simulink model "G474_Mode2_Direct_Start_Repair"  (R2024b)
settings: Solver=FixedStepDiscrete  StartTime=0.0  StopTime=q.stop_time  FixedStep=p.Ts  RelTol=1e-3
InitFcn:
  | m2_project_root=fileparts(fileparts(get_param(bdroot,'FileName')));Simulink.fileGenControl('set','CacheFolder',fullfile(m2_project_root,'work'),'CodeGenFolder',fullfile(m2_project_root,'work'),'createDir',true);m2_ws=get_param(bdroot,'ModelWorkspace');m2_q=getVariable(m2_ws,'q');if isfield(m2_q,'random_initial_angle') && m2_q.random_initial_angle,m2_q.initial_theta_e=2*pi*rand();end;m2_q.initial_state=[0;0;m2_q.initial_rpm*2*pi/60;m2_q.initial_theta_e];assignin(m2_ws,'q',m2_q);fprintf('MODE2 physical initial electrical angle: %.9f deg (random=%d)\n',m2_q.initial_theta_e*180/pi,m2_q.random_initial_angle);
model workspace (MAT data in the model file):
  fSin = [0 0.00153398001567 0.00306795700453 0.00460192607716 0.00613588513806 0.00766982883215 0.00920375529677 0.0107376594096 0.0122715383768 0.0138053894043 0.0153392059729 0.0168729871511 ... (1025 elements, 1025x1)]
  p : object (value not decoded)
  q : object (value not decoded)
  s0 : object (value not decoded)
symbols that are objects in the model workspace (value not decoded): p, q, s0
(part 2 of 2)

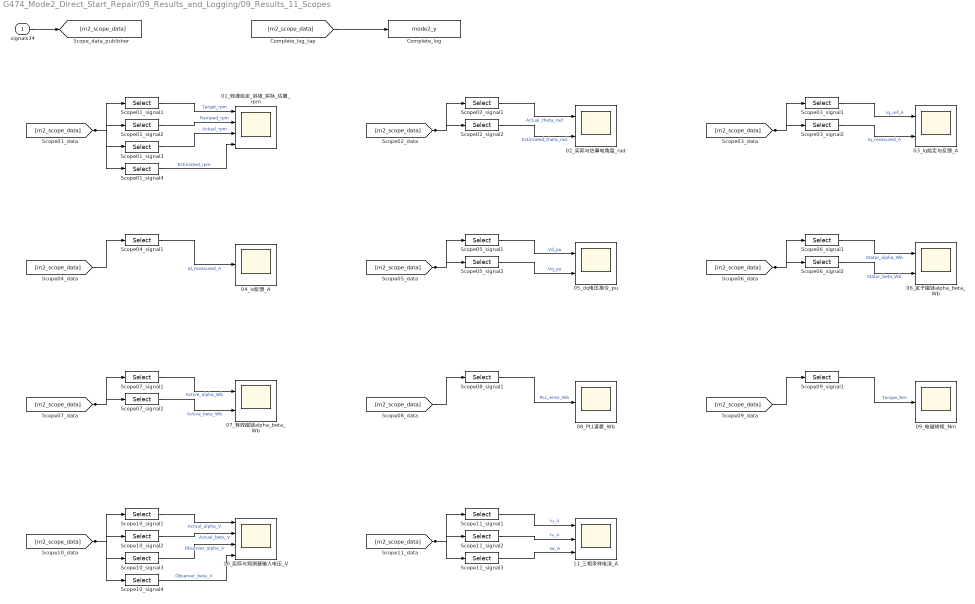
== system G474_Mode2_Direct_Start_Repair/09_Results_and_Logging/09_Results_11_Scopes ==
  signals34 : Inport
  01_转速给定_斜坡_实际_估算_rpm : Scope  NumInputPorts=4
  02_实际与估算电角度_rad : Scope  NumInputPorts=2
  03_Iq给定与反馈_A : Scope  NumInputPorts=2
  04_Id反馈_A : Scope
  05_dq电压指令_pu : Scope  NumInputPorts=2
  06_定子磁链alpha_beta_Wb : Scope  NumInputPorts=2
  07_有效磁链alpha_beta_Wb : Scope  NumInputPorts=2
  08_PLL误差_Wb : Scope
  09_电磁转矩_Nm : Scope
  10_实际与观测器输入电压_V : Scope  NumInputPorts=4
  11_三相采样电流_A : Scope  NumInputPorts=3
  Complete_log : ToWorkspace  VariableName=mode2_y  SaveFormat=Timeseries  SampleTime=-1
  Scope01_signal1 : Selector  InputPortWidth=34  IndexOptions=Index vector (dialog)  Indices=31  OutputSizes=1
  Scope01_signal2 : Selector  InputPortWidth=34  IndexOptions=Index vector (dialog)  Indices=23  OutputSizes=1
  Scope01_signal3 : Selector  InputPortWidth=34  IndexOptions=Index vector (dialog)  Indices=12  OutputSizes=1
  Scope01_signal4 : Selector  InputPortWidth=34  IndexOptions=Index vector (dialog)  Indices=3  OutputSizes=1
  Scope02_signal1 : Selector  InputPortWidth=34  IndexOptions=Index vector (dialog)  Indices=13  OutputSizes=1
  Scope02_signal2 : Selector  InputPortWidth=34  IndexOptions=Index vector (dialog)  Indices=1  OutputSizes=1
  Scope03_signal1 : Selector  InputPortWidth=34  IndexOptions=Index vector (dialog)  Indices=22  OutputSizes=1
  Scope03_signal2 : Selector  InputPortWidth=34  IndexOptions=Index vector (dialog)  Indices=19  OutputSizes=1
  Scope04_signal1 : Selector  InputPortWidth=34  IndexOptions=Index vector (dialog)  Indices=18  OutputSizes=1
  Scope05_signal1 : Selector  InputPortWidth=34  IndexOptions=Index vector (dialog)  Indices=20  OutputSizes=1
  Scope05_signal2 : Selector  InputPortWidth=34  IndexOptions=Index vector (dialog)  Indices=21  OutputSizes=1
  Scope06_signal1 : Selector  InputPortWidth=34  IndexOptions=Index vector (dialog)  Indices=6  OutputSizes=1
  Scope06_signal2 : Selector  InputPortWidth=34  IndexOptions=Index vector (dialog)  Indices=7  OutputSizes=1
  Scope07_signal1 : Selector  InputPortWidth=34  IndexOptions=Index vector (dialog)  Indices=4  OutputSizes=1
  Scope07_signal2 : Selector  InputPortWidth=34  IndexOptions=Index vector (dialog)  Indices=5  OutputSizes=1
  Scope08_signal1 : Selector  InputPortWidth=34  IndexOptions=Index vector (dialog)  Indices=8  OutputSizes=1
  Scope09_signal1 : Selector  InputPortWidth=34  IndexOptions=Index vector (dialog)  Indices=14  OutputSizes=1
  Scope10_signal1 : Selector  InputPortWidth=34  IndexOptions=Index vector (dialog)  Indices=26  OutputSizes=1
  Scope10_signal2 : Selector  InputPortWidth=34  IndexOptions=Index vector (dialog)  Indices=27  OutputSizes=1
  Scope10_signal3 : Selector  InputPortWidth=34  IndexOptions=Index vector (dialog)  Indices=10  OutputSizes=1
  Scope10_signal4 : Selector  InputPortWidth=34  IndexOptions=Index vector (dialog)  Indices=11  OutputSizes=1
  Scope11_signal1 : Selector  InputPortWidth=34  IndexOptions=Index vector (dialog)  Indices=15  OutputSizes=1
  Scope11_signal2 : Selector  InputPortWidth=34  IndexOptions=Index vector (dialog)  Indices=16  OutputSizes=1
  Scope11_signal3 : Selector  InputPortWidth=34  IndexOptions=Index vector (dialog)  Indices=17  OutputSizes=1
  wires:
  signals34/1 -> [m2_scope_data]
  [m2_scope_data] -> Complete_log/1
  [m2_scope_data] -> Scope01_signal1/1, Scope01_signal2/1, Scope01_signal3/1, Scope01_signal4/1
  Scope01_signal1/1 -> 01_转速给定_斜坡_实际_估算_rpm/1  "Target_rpm"
  Scope01_signal2/1 -> 01_转速给定_斜坡_实际_估算_rpm/2  "Ramped_rpm"
  Scope01_signal3/1 -> 01_转速给定_斜坡_实际_估算_rpm/3  "Actual_rpm"
  Scope01_signal4/1 -> 01_转速给定_斜坡_实际_估算_rpm/4  "Estimated_rpm"
  [m2_scope_data] -> Scope02_signal1/1, Scope02_signal2/1
  Scope02_signal1/1 -> 02_实际与估算电角度_rad/1  "Actual_theta_rad"
  Scope02_signal2/1 -> 02_实际与估算电角度_rad/2  "Estimated_theta_rad"
  [m2_scope_data] -> Scope03_signal1/1, Scope03_signal2/1
  Scope03_signal1/1 -> 03_Iq给定与反馈_A/1  "Iq_ref_A"
  Scope03_signal2/1 -> 03_Iq给定与反馈_A/2  "Iq_measured_A"
  [m2_scope_data] -> Scope04_signal1/1
  Scope04_signal1/1 -> 04_Id反馈_A/1  "Id_measured_A"
  [m2_scope_data] -> Scope05_signal1/1, Scope05_signal2/1
  Scope05_signal1/1 -> 05_dq电压指令_pu/1  "Vd_pu"
  Scope05_signal2/1 -> 05_dq电压指令_pu/2  "Vq_pu"
  [m2_scope_data] -> Scope06_signal1/1, Scope06_signal2/1
  Scope06_signal1/1 -> 06_定子磁链alpha_beta_Wb/1  "Stator_alpha_Wb"
  Scope06_signal2/1 -> 06_定子磁链alpha_beta_Wb/2  "Stator_beta_Wb"
  [m2_scope_data] -> Scope07_signal1/1, Scope07_signal2/1
  Scope07_signal1/1 -> 07_有效磁链alpha_beta_Wb/1  "Active_alpha_Wb"
  Scope07_signal2/1 -> 07_有效磁链alpha_beta_Wb/2  "Active_beta_Wb"
  [m2_scope_data] -> Scope08_signal1/1
  Scope08_signal1/1 -> 08_PLL误差_Wb/1  "PLL_error_Wb"
  [m2_scope_data] -> Scope09_signal1/1
  Scope09_signal1/1 -> 09_电磁转矩_Nm/1  "Torque_Nm"
  [m2_scope_data] -> Scope10_signal1/1, Scope10_signal2/1, Scope10_signal3/1, Scope10_signal4/1
  Scope10_signal1/1 -> 10_实际与观测器输入电压_V/1  "Actual_alpha_V"
  Scope10_signal2/1 -> 10_实际与观测器输入电压_V/2  "Actual_beta_V"
  Scope10_signal3/1 -> 10_实际与观测器输入电压_V/3  "Observer_alpha_V"
  Scope10_signal4/1 -> 10_实际与观测器输入电压_V/4  "Observer_beta_V"
  [m2_scope_data] -> Scope11_signal1/1, Scope11_signal2/1, Scope11_signal3/1
  Scope11_signal1/1 -> 11_三相采样电流_A/1  "Iu_A"
  Scope11_signal2/1 -> 11_三相采样电流_A/2  "Iv_A"
  Scope11_signal3/1 -> 11_三相采样电流_A/3  "Iw_A"

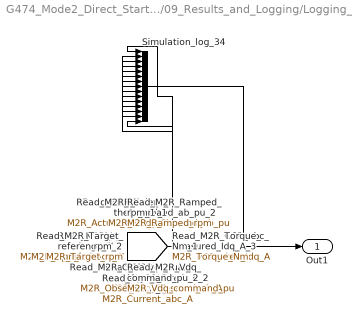
== system G474_Mode2_Direct_Start_Repair/09_Results_and_Logging/Logging_taps ==
  Simulation_log_34 : Mux  Inputs=15
  Out1 : Outport
  wires:
  [M2R_Actual_theta_rad] -> Simulation_log_34/3
  [M2R_Actual_rpm] -> Simulation_log_34/2
  [M2R_Torque_Nm] -> Simulation_log_34/4
  [M2R_CCR_abc] -> Simulation_log_34/12
  [M2R_Command_ab_pu] -> Simulation_log_34/10
  [M2R_Current_abc_A] -> Simulation_log_34/5
  [M2R_Observer_y11] -> Simulation_log_34/1
  [M2R_Iq_reference_A] -> Simulation_log_34/8
  Simulation_log_34/1 -> Out1/1
  [M2R_Vdq_command_pu] -> Simulation_log_34/7
  [M2R_Measured_Idq_A] -> Simulation_log_34/6
  [M2R_Measured_ab_A] -> Simulation_log_34/15
  [M2R_Bridge_voltage_V] -> Simulation_log_34/11
  [M2R_Target_rpm] -> Simulation_log_34/13
  [M2R_Mode_2] -> Simulation_log_34/14
  [M2R_Ramped_rpm] -> Simulation_log_34/9

== system G474_Mode2_Direct_Start_Repair/03_Hybrid_Flux_Observer/02_Active_Flux_Models/Current model ==
  theta_previous : Inport
  Id : Inport  Port=2
  Active scalar : Sum
  Cos : Trigonometry  Operator=cos
  Direction : Mux  Inputs=2
  PM flux : Constant  Value=p.Flux
  Projection : Product  Inputs=**
  Saliency : Gain  Gain=p.Ld-p.Lq
  Sin : Trigonometry
  psi_I : Outport
  wires:
  Projection/1 -> psi_I/1
  Sin/1 -> Direction/2
  Active scalar/1 -> Projection/1
  Cos/1 -> Direction/1
  Saliency/1 -> Active scalar/2
  PM flux/1 -> Active scalar/1
  theta_previous/1 -> Cos/1, Sin/1
  Direction/1 -> Projection/2
  Id/1 -> Saliency/1

== system G474_Mode2_Direct_Start_Repair/03_Hybrid_Flux_Observer/02_Active_Flux_Models/Voltage model extraction ==
  psi_s_previous : Inport
  current_ab : Inport  Port=2
  Active flux : Sum  Inputs=+-
  Inductive flux : Gain  Gain=p.Lq
  psi_V : Outport
  wires:
  Active flux/1 -> psi_V/1
  Inductive flux/1 -> Active flux/2
  psi_s_previous/1 -> Active flux/1
  current_ab/1 -> Inductive flux/1

== system G474_Mode2_Direct_Start_Repair/03_Hybrid_Flux_Observer/03_Flux_Feedback/Alpha_PI ==
  note: flux.c: Comp_Interg += error*Comp_Ki; Ucomp = error*Comp_Kp + Comp_Interg.
      | No integral/output saturation in this firmware branch. SMO selection freezes PI memory.
  error : Inport
  integral_enable : Inport  Port=2
  Enable_integral : Switch  Criteria=u2 ~= 0  SaturateOnIntegerOverflow=off  InputSameDT=off
  Integral_candidate : Sum
  Integral_increment : Gain  Gain=Ki
  Pre_output : Sum
  Previous_integral : UnitDelay  SampleTime=Ts  HasFrameUpgradeWarning=on
  Proportional : Gain  Gain=Kp
  Ucomp : Outport
  integral : Outport  Port=2
  wires:
  Pre_output/1 -> Ucomp/1
  Proportional/1 -> Pre_output/1
  integral_enable/1 -> Enable_integral/2
  Integral_candidate/1 -> Enable_integral/1
  Previous_integral/1 -> Integral_candidate/1, Enable_integral/3
  Integral_increment/1 -> Integral_candidate/2
  Enable_integral/1 -> Previous_integral/1, integral/1, Pre_output/2
  error/1 -> Integral_increment/1, Proportional/1

== system G474_Mode2_Direct_Start_Repair/03_Hybrid_Flux_Observer/03_Flux_Feedback/Beta_PI ==
  note: flux.c: Comp_Interg += error*Comp_Ki; Ucomp = error*Comp_Kp + Comp_Interg.
      | No integral/output saturation in this firmware branch. SMO selection freezes PI memory.
  error : Inport
  integral_enable : Inport  Port=2
  Enable_integral : Switch  Criteria=u2 ~= 0  SaturateOnIntegerOverflow=off  InputSameDT=off
  Integral_candidate : Sum
  Integral_increment : Gain  Gain=Ki
  Pre_output : Sum
  Previous_integral : UnitDelay  SampleTime=Ts  HasFrameUpgradeWarning=on
  Proportional : Gain  Gain=Kp
  Ucomp : Outport
  integral : Outport  Port=2
  wires:
  Pre_output/1 -> Ucomp/1
  Proportional/1 -> Pre_output/1
  integral_enable/1 -> Enable_integral/2
  Integral_candidate/1 -> Enable_integral/1
  Previous_integral/1 -> Integral_candidate/1, Enable_integral/3
  Integral_increment/1 -> Integral_candidate/2
  Enable_integral/1 -> Previous_integral/1, integral/1, Pre_output/2
  error/1 -> Integral_increment/1, Proportional/1

== system G474_Mode2_Direct_Start_Repair/03_Hybrid_Flux_Observer/03_Flux_Feedback/SMO_feedback ==
  In1 : Inport
  Boundary normalization : Gain  Gain=1/p.SMO_Boundary
  Boundary saturation : Saturate  UpperLimit=1  LowerLimit=-1
  Sliding gain : Gain  Gain=p.SMO_Kslide
  Out1 : Outport
  wires:
  Sliding gain/1 -> Out1/1
  Boundary saturation/1 -> Sliding gain/1
  In1/1 -> Boundary normalization/1
  Boundary normalization/1 -> Boundary saturation/1

== system G474_Mode2_Direct_Start_Repair/03_Hybrid_Flux_Observer/05_PLL_and_Angle/PLL ==
  psi_V : Inport
  theta_previous : Inport  Port=2
  Angle_update : Subsystem
      settings: OpenFcn=open_system(gcb,'force')
      mask Display: port_label('input',1,'In1');port_label('input',2,'In2');port_label('output',1,'Out1');
  PLL_PI : Subsystem  mask{Kp=p.PLL_kp, Ki=p.PLL_ki, Ts=p.Ts}
      mask prompts: Kp "Kp (source coefficient)"; Ki "Ki (per call, already discrete)"; Ts "Execution period (s)"
      settings: OpenFcn=open_system(gcb,'force')
      mask Display: port_label('input',1,'PLL_Err');port_label('input',2,'step_limit');port_label('output',1,'PLL_Ui');port_label('output',2,'PLL_Interg');
  Phase_detector : Subsystem
      settings: OpenFcn=open_system(gcb,'force')
      mask Display: port_label('input',1,'In1');port_label('input',2,'In2');port_label('output',1,'Out1');
  Step limit value : Constant  Value=p.pll_step_limit
  theta_new : Outport
  step_rad : Outport  Port=2
  PLL_error : Outport  Port=3
  wires:
  Angle_update/1(Out1) -> theta_new/1
  Step limit value/1 -> PLL_PI/2(step_limit)
  Phase_detector/1(Out1) -> PLL_error/1, PLL_PI/1(PLL_Err)
  PLL_PI/1(PLL_Ui) -> Angle_update/2(In2), step_rad/1
  theta_previous/1 -> Angle_update/1(In1), Phase_detector/2(In2)
  psi_V/1 -> Phase_detector/1(In1)

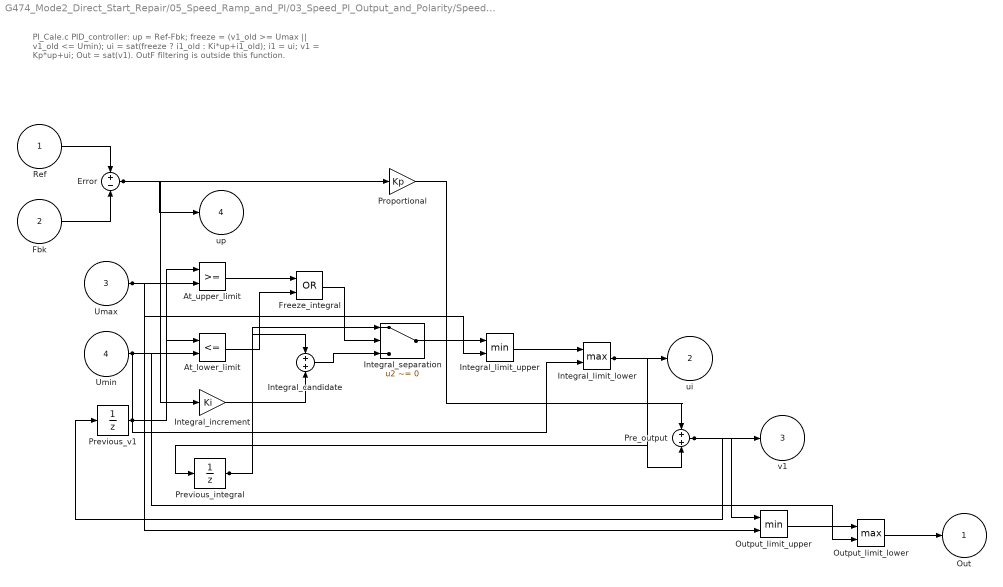
== system G474_Mode2_Direct_Start_Repair/05_Speed_Ramp_and_PI/03_Speed_PI_Output_and_Polarity/Speed_PI ==
  note: PI_Cale.c PID_controller:
      | up = Ref-Fbk; freeze = (v1_old >= Umax || v1_old <= Umin);
      | ui = sat(freeze ? i1_old : Ki*up+i1_old); i1 = ui;
      | v1 = Kp*up+ui; Out = sat(v1). OutF filtering is outside this function.
  Ref : Inport
  Fbk : Inport  Port=2
  Umax : Inport  Port=3
  Umin : Inport  Port=4
  At_lower_limit : RelationalOperator  Operator=<=  OutDataTypeStr=boolean  RndMeth=Simplest  InputSameDT=off
  At_upper_limit : RelationalOperator  OutDataTypeStr=boolean  RndMeth=Simplest  InputSameDT=off
  Error : Sum  Inputs=+-
  Freeze_integral : Logic  Operator=OR  AllPortsSameDT=off  OutDataTypeStr=boolean
  Integral_candidate : Sum
  Integral_increment : Gain  Gain=Ki
  Integral_limit_lower : MinMax  Function=max  Inputs=2
  Integral_limit_upper : MinMax  Inputs=2
  Integral_separation : Switch  Criteria=u2 ~= 0  SaturateOnIntegerOverflow=off  InputSameDT=off
  Output_limit_lower : MinMax  Function=max  Inputs=2
  Output_limit_upper : MinMax  Inputs=2
  Pre_output : Sum
  Previous_integral : UnitDelay  SampleTime=Ts  HasFrameUpgradeWarning=on
  Previous_v1 : UnitDelay  SampleTime=Ts  HasFrameUpgradeWarning=on
  Proportional : Gain  Gain=Kp
  Out : Outport
  ui : Outport  Port=2
  v1 : Outport  Port=3
  up : Outport  Port=4
  wires:
  Umax/1 -> Output_limit_upper/2, Integral_limit_upper/2, At_upper_limit/2
  Ref/1 -> Error/1
  At_lower_limit/1 -> Freeze_integral/2
  Error/1 -> Proportional/1, Integral_increment/1, up/1
  Fbk/1 -> Error/2
  At_upper_limit/1 -> Freeze_integral/1
  Umin/1 -> Integral_limit_lower/2, Output_limit_lower/2, At_lower_limit/2
  Previous_v1/1 -> At_upper_limit/1, At_lower_limit/1
  Integral_increment/1 -> Integral_candidate/2
  Previous_integral/1 -> Integral_candidate/1, Integral_separation/1
  Freeze_integral/1 -> Integral_separation/2
  Integral_candidate/1 -> Integral_separation/3
  Proportional/1 -> Pre_output/1
  Integral_separation/1 -> Integral_limit_upper/1
  Integral_limit_upper/1 -> Integral_limit_lower/1
  Integral_limit_lower/1 -> Pre_output/2, ui/1, Previous_integral/1
  Pre_output/1 -> Previous_v1/1, Output_limit_upper/1, v1/1
  Output_limit_upper/1 -> Output_limit_lower/1
  Output_limit_lower/1 -> Out/1

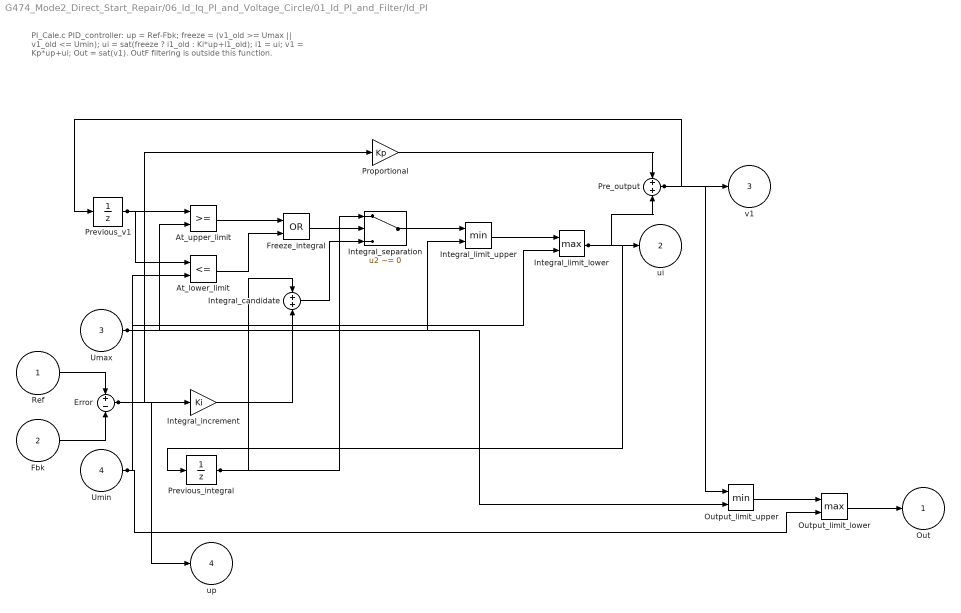
== system G474_Mode2_Direct_Start_Repair/06_Id_Iq_PI_and_Voltage_Circle/01_Id_PI_and_Filter/Id_PI ==
  note: PI_Cale.c PID_controller:
      | up = Ref-Fbk; freeze = (v1_old >= Umax || v1_old <= Umin);
      | ui = sat(freeze ? i1_old : Ki*up+i1_old); i1 = ui;
      | v1 = Kp*up+ui; Out = sat(v1). OutF filtering is outside this function.
  Ref : Inport
  Fbk : Inport  Port=2
  Umax : Inport  Port=3
  Umin : Inport  Port=4
  At_lower_limit : RelationalOperator  Operator=<=  OutDataTypeStr=boolean  RndMeth=Simplest  InputSameDT=off
  At_upper_limit : RelationalOperator  OutDataTypeStr=boolean  RndMeth=Simplest  InputSameDT=off
  Error : Sum  Inputs=+-
  Freeze_integral : Logic  Operator=OR  AllPortsSameDT=off  OutDataTypeStr=boolean
  Integral_candidate : Sum
  Integral_increment : Gain  Gain=Ki
  Integral_limit_lower : MinMax  Function=max  Inputs=2
  Integral_limit_upper : MinMax  Inputs=2
  Integral_separation : Switch  Criteria=u2 ~= 0  SaturateOnIntegerOverflow=off  InputSameDT=off
  Output_limit_lower : MinMax  Function=max  Inputs=2
  Output_limit_upper : MinMax  Inputs=2
  Pre_output : Sum
  Previous_integral : UnitDelay  SampleTime=Ts  HasFrameUpgradeWarning=on
  Previous_v1 : UnitDelay  SampleTime=Ts  HasFrameUpgradeWarning=on
  Proportional : Gain  Gain=Kp
  Out : Outport
  ui : Outport  Port=2
  v1 : Outport  Port=3
  up : Outport  Port=4
  wires:
  Umax/1 -> Output_limit_upper/2, Integral_limit_upper/2, At_upper_limit/2
  Previous_v1/1 -> At_lower_limit/1, At_upper_limit/1
  Ref/1 -> Error/1
  At_lower_limit/1 -> Freeze_integral/2
  Error/1 -> Proportional/1, Integral_increment/1, up/1
  Fbk/1 -> Error/2
  At_upper_limit/1 -> Freeze_integral/1
  Umin/1 -> Integral_limit_lower/2, Output_limit_lower/2, At_lower_limit/2
  Integral_increment/1 -> Integral_candidate/2
  Previous_integral/1 -> Integral_candidate/1, Integral_separation/1
  Freeze_integral/1 -> Integral_separation/2
  Integral_candidate/1 -> Integral_separation/3
  Proportional/1 -> Pre_output/1
  Integral_separation/1 -> Integral_limit_upper/1
  Integral_limit_upper/1 -> Integral_limit_lower/1
  Integral_limit_lower/1 -> Previous_integral/1, Pre_output/2, ui/1
  Pre_output/1 -> Previous_v1/1, Output_limit_upper/1, v1/1
  Output_limit_upper/1 -> Output_limit_lower/1
  Output_limit_lower/1 -> Out/1

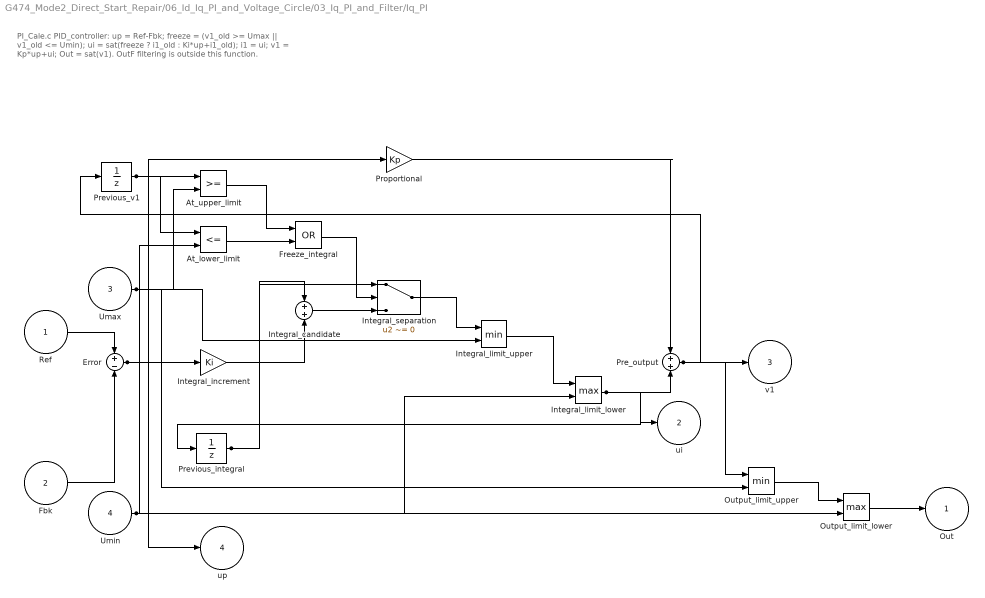
== system G474_Mode2_Direct_Start_Repair/06_Id_Iq_PI_and_Voltage_Circle/03_Iq_PI_and_Filter/Iq_PI ==
  note: PI_Cale.c PID_controller:
      | up = Ref-Fbk; freeze = (v1_old >= Umax || v1_old <= Umin);
      | ui = sat(freeze ? i1_old : Ki*up+i1_old); i1 = ui;
      | v1 = Kp*up+ui; Out = sat(v1). OutF filtering is outside this function.
  Ref : Inport
  Fbk : Inport  Port=2
  Umax : Inport  Port=3
  Umin : Inport  Port=4
  At_lower_limit : RelationalOperator  Operator=<=  OutDataTypeStr=boolean  RndMeth=Simplest  InputSameDT=off
  At_upper_limit : RelationalOperator  OutDataTypeStr=boolean  RndMeth=Simplest  InputSameDT=off
  Error : Sum  Inputs=+-
  Freeze_integral : Logic  Operator=OR  AllPortsSameDT=off  OutDataTypeStr=boolean
  Integral_candidate : Sum
  Integral_increment : Gain  Gain=Ki
  Integral_limit_lower : MinMax  Function=max  Inputs=2
  Integral_limit_upper : MinMax  Inputs=2
  Integral_separation : Switch  Criteria=u2 ~= 0  SaturateOnIntegerOverflow=off  InputSameDT=off
  Output_limit_lower : MinMax  Function=max  Inputs=2
  Output_limit_upper : MinMax  Inputs=2
  Pre_output : Sum
  Previous_integral : UnitDelay  SampleTime=Ts  HasFrameUpgradeWarning=on
  Previous_v1 : UnitDelay  SampleTime=Ts  HasFrameUpgradeWarning=on
  Proportional : Gain  Gain=Kp
  Out : Outport
  ui : Outport  Port=2
  v1 : Outport  Port=3
  up : Outport  Port=4
  wires:
  Output_limit_upper/1 -> Output_limit_lower/1
  Pre_output/1 -> Output_limit_upper/1, Previous_v1/1, v1/1
  Integral_limit_lower/1 -> ui/1, Pre_output/2, Previous_integral/1
  Integral_limit_upper/1 -> Integral_limit_lower/1
  Integral_separation/1 -> Integral_limit_upper/1
  Proportional/1 -> Pre_output/1
  Integral_candidate/1 -> Integral_separation/3
  Freeze_integral/1 -> Integral_separation/2
  Output_limit_lower/1 -> Out/1
  Previous_integral/1 -> Integral_separation/1, Integral_candidate/1
  Integral_increment/1 -> Integral_candidate/2
  Error/1 -> Integral_increment/1, up/1, Proportional/1
  At_upper_limit/1 -> Freeze_integral/1
  Previous_v1/1 -> At_lower_limit/1, At_upper_limit/1
  Umax/1 -> At_upper_limit/2, Output_limit_upper/2, Integral_limit_upper/2
  Fbk/1 -> Error/2
  Umin/1 -> Output_limit_lower/2, At_lower_limit/2, Integral_limit_lower/2
  Ref/1 -> Error/1
  At_lower_limit/1 -> Freeze_integral/2

== system G474_Mode2_Direct_Start_Repair/03_Hybrid_Flux_Observer/05_PLL_and_Angle/PLL/Angle_update ==
  In1 : Inport
  In2 : Inport  Port=2
  Angle update : Sum
  Two pi : Constant  Value=2*pi
  Wrap 2pi : Math  Operator=mod
  Out1 : Outport
  wires:
  In1/1 -> Angle update/1
  Wrap 2pi/1 -> Out1/1
  Angle update/1 -> Wrap 2pi/1
  In2/1 -> Angle update/2
  Two pi/1 -> Wrap 2pi/2

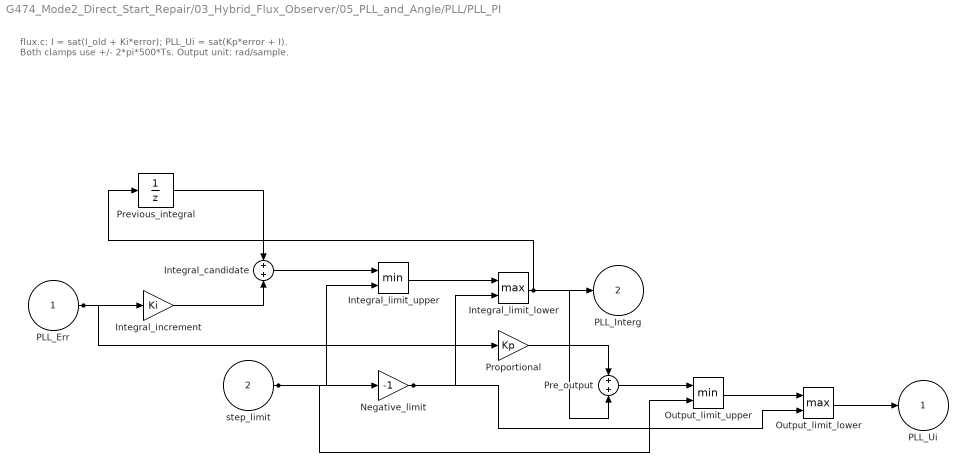
== system G474_Mode2_Direct_Start_Repair/03_Hybrid_Flux_Observer/05_PLL_and_Angle/PLL/PLL_PI ==
  note: flux.c: I = sat(I_old + Ki*error); PLL_Ui = sat(Kp*error + I).
      | Both clamps use +/- 2*pi*500*Ts. Output unit: rad/sample.
  PLL_Err : Inport
  step_limit : Inport  Port=2
  Integral_candidate : Sum
  Integral_increment : Gain  Gain=Ki
  Integral_limit_lower : MinMax  Function=max  Inputs=2
  Integral_limit_upper : MinMax  Inputs=2
  Negative_limit : Gain  Gain=-1
  Output_limit_lower : MinMax  Function=max  Inputs=2
  Output_limit_upper : MinMax  Inputs=2
  Pre_output : Sum
  Previous_integral : UnitDelay  SampleTime=Ts  HasFrameUpgradeWarning=on
  Proportional : Gain  Gain=Kp
  PLL_Ui : Outport
  PLL_Interg : Outport  Port=2
  wires:
  Output_limit_lower/1 -> PLL_Ui/1
  Output_limit_upper/1 -> Output_limit_lower/1
  Pre_output/1 -> Output_limit_upper/1
  Proportional/1 -> Pre_output/1
  Negative_limit/1 -> Integral_limit_lower/2, Output_limit_lower/2
  Integral_limit_upper/1 -> Integral_limit_lower/1
  Integral_candidate/1 -> Integral_limit_upper/1
  Integral_limit_lower/1 -> Previous_integral/1, PLL_Interg/1, Pre_output/2
  Integral_increment/1 -> Integral_candidate/2
  Previous_integral/1 -> Integral_candidate/1
  step_limit/1 -> Integral_limit_upper/2, Negative_limit/1, Output_limit_upper/2
  PLL_Err/1 -> Proportional/1, Integral_increment/1

== system G474_Mode2_Direct_Start_Repair/03_Hybrid_Flux_Observer/05_PLL_and_Angle/PLL/Phase_detector ==
  In1 : Inport
  In2 : Inport  Port=2
  Alpha sin : Product  Inputs=**
  Beta cos : Product  Inputs=**
  Cos : Trigonometry  Operator=cos
  Flux components : Demux  Outputs=2
  Phase error : Sum  Inputs=+-
  Sin : Trigonometry
  Out1 : Outport
  wires:
  Phase error/1 -> Out1/1
  Cos/1 -> Beta cos/2
  Alpha sin/1 -> Phase error/2
  Flux components/2 -> Beta cos/1
  Flux components/1 -> Alpha sin/1
  Sin/1 -> Alpha sin/2
  In2/1 -> Cos/1, Sin/1
  Beta cos/1 -> Phase error/1
  In1/1 -> Flux components/1

== matlab function G474_Mode2_Direct_Start_Repair/04_Clarke_Park/Source_lookup_and_transform ==
  data: iabc input size=[3 1]; dq output size=[2 1]; theta input size=1; iab output size=[2 1]; cs output size=[2 1]; fSin parameter
function [dq,iab,cs]=firmware_park(iabc,theta,fSin)
% Foc.c CURRENT_USE_W_AS_V=0, CURRENT_BETA_SIGN=1, PARK_ANGLE_REVERSE=0.
iab=[iabc(1);(iabc(1)+2*iabc(2))*0.577350269];
angle=fix(651.8986*theta);
if angle>4095, angle=angle-4096; elseif angle<0, angle=angle+4096; end
angle=mod(angle,4096); sector=floor(angle/1024);
% Preserve the original quarter-wave table indices, including 0x3FF offsets.
switch sector
    case 0
        s=fSin(angle+1); c=fSin(1023-angle+1);
    case 1
        s=fSin(2048-angle+1); c=-fSin(angle-1023+1);
    case 2
        s=-fSin(angle-2048+1); c=-fSin(3072-angle+1);
    otherwise
        s=-fSin(4096-angle+1); c=fSin(angle-3072+1);
end
cs=[c;s]; dq=[iab(1)*c+iab(2)*s;iab(2)*c-iab(1)*s];
end

== matlab function G474_Mode2_Direct_Start_Repair/02_PWM_Voltage_and_Current_Sampling/01_PWM_CCR_Applied_Voltage ==
  data: old_command input size=[2 1]; voltage output size=[2 1]; old_ab input size=[2 1]; q parameter
function voltage=reconstruct_voltage(old_command,old_ab,q)
% Known PWM command + previous measured current; no physical plant feedback.
old_phase=[old_ab(1);-0.5*old_ab(1)+sqrt(3)/2*old_ab(2);-0.5*old_ab(1)-sqrt(3)/2*old_ab(2)];
observer=q; observer.actual_deadtime_V=q.observer_deadtime_V;
[voltage,~]=firmware_svpwm(old_command,old_phase,observer);
end

function [voltage,ccr]=firmware_svpwm(command,iabc,q)
% Original sector logic and CCR truncation/clamp; reconstruct average voltages.
a=command(1); b=command(2);
t1=b; t2=b*0.5+a*0.8660254; t3=t2-t1;
sector=3;
if t2>0, sector=sector-1; end
if t3>0, sector=sector-1; end
if t1<0, sector=7-sector; end
if sector==1 || sector==4
    t=[t2;t1-t3;-t2];
elseif sector==2 || sector==5
    t=[t3+t2;t1;-t1];
elseif sector==3 || sector==6
    t=[t3;-t3;-(t1+t2)];
else
    t=zeros(3,1);
end
km=1;
if q.Vbus>1, km=min(max(12/q.Vbus,0.7),1.3); end
ccr=min(max(fix(t*km*2000)+2000,0),3999);
phase=ccr/4000*q.Vbus;
% Plant deadtime is an explicit physical assumption, independently configurable.
physical_i=iabc/q.current_channel_sign;
sgn=double(physical_i>0.01)-double(physical_i< -0.01);
phase=phase-q.actual_deadtime_V*sgn;
voltage=[(2*phase(1)-phase(2)-phase(3))/3;(phase(2)-phase(3))/sqrt(3)];
end

== matlab function G474_Mode2_Direct_Start_Repair/07_InversePark_SVPWM_Inverter/Inverse_Park ==
  data: vdq input size=[2 1]; command output size=[2 1]; cs input size=[2 1]
function command=firmware_inverse_park(vdq,cs)
command=[vdq(1)*cs(1)-vdq(2)*cs(2);vdq(2)*cs(1)+vdq(1)*cs(2)];
end

== matlab function G474_Mode2_Direct_Start_Repair/07_InversePark_SVPWM_Inverter/Source_SVPWM_and_average_bridge ==
  data: command input size=[2 1]; voltage output size=[2 1]; iabc input size=[3 1]; ccr output size=[3 1]; q parameter
function [voltage,ccr]=firmware_svpwm(command,iabc,q)
% Original sector logic and CCR truncation/clamp; reconstruct average voltages.
a=command(1); b=command(2);
t1=b; t2=b*0.5+a*0.8660254; t3=t2-t1;
sector=3;
if t2>0, sector=sector-1; end
if t3>0, sector=sector-1; end
if t1<0, sector=7-sector; end
if sector==1 || sector==4
    t=[t2;t1-t3;-t2];
elseif sector==2 || sector==5
    t=[t3+t2;t1;-t1];
elseif sector==3 || sector==6
    t=[t3;-t3;-(t1+t2)];
else
    t=zeros(3,1);
end
km=1;
if q.Vbus>1, km=min(max(12/q.Vbus,0.7),1.3); end
ccr=min(max(fix(t*km*2000)+2000,0),3999);
phase=ccr/4000*q.Vbus;
% Plant deadtime is an explicit physical assumption, independently configurable.
physical_i=iabc/q.current_channel_sign;
sgn=double(physical_i>0.01)-double(physical_i< -0.01);
phase=phase-q.actual_deadtime_V*sgn;
voltage=[(2*phase(1)-phase(2)-phase(3))/3;(phase(2)-phase(3))/sqrt(3)];
end

== matlab function G474_Mode2_Direct_Start_Repair/07_InversePark_SVPWM_Inverter/Deadtime_Voltage_Feedforward ==
  data: desired_command input size=[2 1]; applied_command output size=[2 1]; phase_i input size=[3 1]; estimated_rpm input size=1; time input size=1; q parameter
function applied_command=deadtime_feedforward(desired_command,phase_i,estimated_rpm,time,q)
% Inverter voltage feedforward using measured phase-current polarity.
% This compensates physical voltage loss, not the displayed torque signal.
km=min(max(12/q.Vbus,0.7),1.3);
polarity=double(phase_i>0.01)-double(phase_i< -0.01);
time_gate=min(max((time-q.feedforward_start_s)/q.feedforward_ramp_s,0),1);
speed_gate=min(max((abs(estimated_rpm)-80)/80,0),1);
loss=time_gate*speed_gate*q.deadtime_feedforward_V*[(2*polarity(1)-polarity(2)-polarity(3))/3; ...
    (polarity(2)-polarity(3))/sqrt(3)];
applied_command=desired_command+sqrt(3)/(q.Vbus*km)*loss;
end

== matlab function G474_Mode2_Direct_Start_Repair/08_PMSM_Electrical_Mechanical_Plant/Electrical_and_mechanical_RK4 ==
  data: x input size=[4 1]; xn output size=[4 1]; v input size=[2 1]; q parameter
function xn=pmsm_rk4(x,v,q)
% Four RK4 substeps per PWM period; electrical/mechanical model, not firmware.
xn=x; h=q.Ts/4;
for k=1:4
    a=rhs(xn,v,q); b=rhs(xn+h*a/2,v,q);
    c=rhs(xn+h*b/2,v,q); d=rhs(xn+h*c,v,q);
    xn=xn+h*(a+2*b+2*c+d)/6;
end
xn(4)=mod(xn(4),2*pi);
end
function dx=rhs(x,v,q)
c=cos(x(4)); s=sin(x(4)); we=q.pole_pairs*x(3);
vd=v(1)*c+v(2)*s; vq=-v(1)*s+v(2)*c;
te=1.5*q.pole_pairs*(q.Flux*x(2)+(q.Ld-q.Lq)*x(1)*x(2));
load=q.load_torque;
if isfield(q,'load_speed_scale_rad_s') && q.load_speed_scale_rad_s>0
    load=q.load_torque*tanh(x(3)/q.load_speed_scale_rad_s);
end
dx=[(vd-q.Rs*x(1)+we*q.Lq*x(2))/q.Ld; ...
    (vq-q.Rs*x(2)-we*(q.Ld*x(1)+q.Flux))/q.Lq; ...
    (te-q.B*x(3)-load)/q.J; we];
end

== matlab function G474_Mode2_Direct_Start_Repair/08_PMSM_Electrical_Mechanical_Plant/Physical_measurements ==
  data: x input size=[4 1]; iabc output size=[3 1]; iab output size=[2 1]; rpm output size=1; theta output size=1; torque output size=1; q parameter
function [iabc,iab,rpm,theta,torque]=phase_measurements(x,q)
% Averaged physical PMSM measurements. True angle never enters controller.
c=cos(x(4)); s=sin(x(4));
iab=[x(1)*c-x(2)*s;x(1)*s+x(2)*c];
iabc=[iab(1);-0.5*iab(1)+sqrt(3)/2*iab(2);-0.5*iab(1)-sqrt(3)/2*iab(2)];
iabc=q.current_channel_sign*iabc;
rpm=x(3)*60/(2*pi); theta=mod(x(4),2*pi);
torque=1.5*q.pole_pairs*(q.Flux*x(2)+(q.Ld-q.Lq)*x(1)*x(2));
end
